simulink model "dcmotor_20240522"  (R2022a)
settings: Solver=ode45  StartTime=0.0  StopTime=1  RelTol=1e-3
values from neighbouring files (symbols this model uses):
  Ce = 1/317    (= 0.00315457413249)    [init_dc_servo.m]
  Cm = 30.2e-3    (= 0.0302)    [init_dc_servo.m]
  J = 142e-7    (= 1.42e-05)    [init_dc_servo.m]
  Kii = 600    [init_dc_servo.m]
  Kip = 2700    [init_dc_servo.m]
  Kpp = 30    [init_dc_servo.m]
  Kvi = 60    [init_dc_servo.m]
  Kvp = 1200    [init_dc_servo.m]
  L = 0.0823e-3    (= 8.23e-05)    [init_dc_servo.m]
  R = 0.299    [init_dc_servo.m]    (also in para_for_math_pmsm.m = 0.958)
libraries: simulink_extras x17, spspowerguiLib x1
settings Model: Creator=ccaao  LastModifiedBy=ccaao

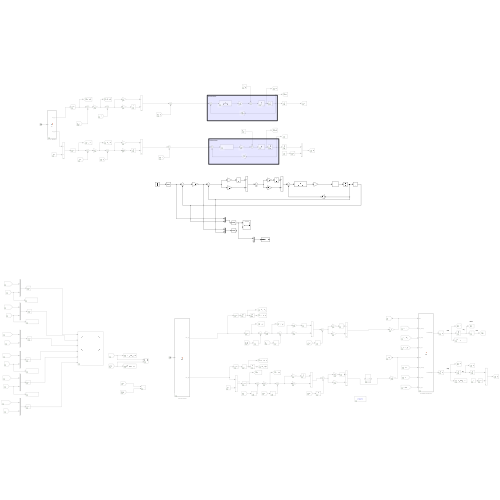
[thumbnail: Simulink's stored preview of the top-level diagram]
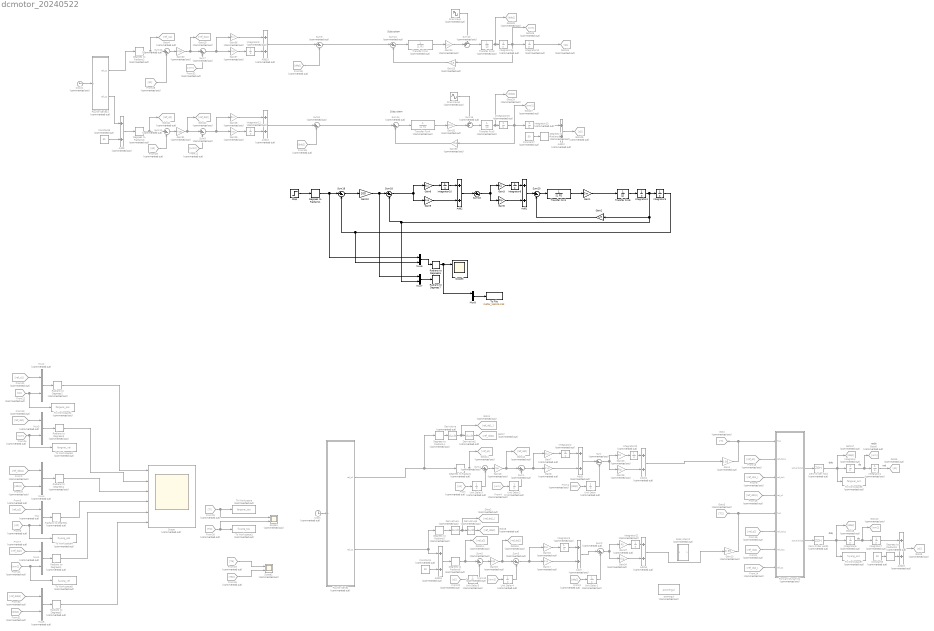
== system dcmotor_20240522 ==
  note: Subsystem
  note: rad/s
  note: rad
  note: dq
  note: ddq
  note: dq
  note: ddq
  note: Subsystem
  Add1 : Sum
  Add{3,7,9..14,18..19} (10 alike) : Sum  Commented=on
  Add2 : Sum
  Clock : Clock  Commented=on
  Clock1 : Clock  Commented=on
  Constant{4..7} (4 alike) : Constant  Commented=on  Value=50
  Degrees to Radians{,2..6,8..9} (8 alike) : simulink_extras/Transformations/Degrees to Radians  Commented=on
  Degrees to Radians1 : simulink_extras/Transformations/Degrees to Radians
  Derivative{,1..3} (4 alike) : Derivative  Commented=on
  Forward Dynamics : MATLAB Function  Commented=on  TreatAsAtomicUnit=on
  Fourier Series : MATLAB Function  Commented=on  TreatAsAtomicUnit=on
  Fourier Series1 : MATLAB Function  Commented=on  TreatAsAtomicUnit=on
  From : From  Commented=on  GotoTag=q1
  From1 : From  Commented=on  GotoTag=ddq1
  From10 : From  Commented=on  GotoTag=wm2
  From11 : From  Commented=on  GotoTag=wm2
  From12 : From  Commented=on  GotoTag=wm2
  From13 : From  Commented=on  GotoTag=ref_q1
  From14 : From  Commented=on  GotoTag=ref_dq2_
  From15 : From  Commented=on  GotoTag=ref_ddq1
  From16 : From  Commented=on  GotoTag=ref_q2
  From19 : From  Commented=on  GotoTag=Te
  From2 : From  Commented=on  GotoTag=ref_ddq1
  From20 : From  Commented=on  GotoTag=q2
  From21 : From  Commented=on  GotoTag=ref_q1
  From22 : From  Commented=on  GotoTag=q1
  From23 : From  Commented=on  GotoTag=ref_dq1
  From24 : From  Commented=on  GotoTag=wm
  From25 : From  Commented=on  GotoTag=Tl
  From26 : From  Commented=on  GotoTag=Tl2
  From27 : From  Commented=on  GotoTag=ddq1
  From28 : From  Commented=on  GotoTag=q1
  From29 : From  Commented=on  GotoTag=q2
  From3 : From  Commented=on  GotoTag=ddq2
  From30 : From  Commented=on  GotoTag=ref_ddq2
  From31 : From  Commented=on  GotoTag=ddq2
  From32 : From  Commented=on  GotoTag=wm
  From35 : From  Commented=on  GotoTag=ddq1
  From36 : From  Commented=on  GotoTag=ddq2
  From4 : From  Commented=on  GotoTag=wm
  From45 : From  Commented=on  GotoTag=Te2
  From5 : From  Commented=on  GotoTag=ref_q2
  From6 : From  Commented=on  GotoTag=q2
  From7 : From  Commented=on  GotoTag=ref_dq2
  From8 : From  Commented=on  GotoTag=ref_dq1_
  From9 : From  Commented=on  GotoTag=ref_dq2
  Gain1 : Gain  Gain=Cm
  Gain10 : Gain  Gain=100
  Gain13 : Gain  Commented=on  Gain=0.95
  Gain{7,16,28,36} (4 alike) : Gain  Commented=on  Gain=Kvi
  Gain{8,17,29,37} (4 alike) : Gain  Commented=on  Gain=Kvp
  Gain{18..19,30..31} (4 alike) : Gain  Commented=on  Gain=Kpp
  Gain2 : Gain  Gain=Ce
  Gain23 : Gain  Commented=on  Gain=Kii
  Gain24 : Gain  Commented=on  Gain=Cm
  Gain25 : Gain  Commented=on  Gain=Ce
  Gain26 : Gain  Commented=on  Gain=Kip
  Gain27 : Gain  Commented=on  Gain=Kii
  Gain3 : Gain  Gain=Kii
  Gain32 : Gain  Commented=on  Gain=Cm
  Gain33 : Gain  Commented=on  Gain=Ce
  Gain34 : Gain  Commented=on  Gain=Kip
  Gain4 : Gain  Commented=on  Gain=0.95
  Gain5 : Gain  Gain=Kip
  Gain6 : Gain  Gain=Kvi
  Gain9 : Gain  Gain=Kvp
  Goto : Goto  Commented=on  GotoTag=Tl
  Goto1 : Goto  Commented=on  GotoTag=ref_dq1_
  Goto10 : Goto  Commented=on  GotoTag=wm2
  Goto11 : Goto  Commented=on  GotoTag=ref_q1
  Goto12 : Goto  Commented=on  GotoTag=ref_dq1
  Goto14 : Goto  Commented=on  GotoTag=ref_q2
  Goto15 : Goto  Commented=on  GotoTag=ref_dq2
  Goto17 : Goto  Commented=on  GotoTag=ddq1
  Goto18 : Goto  Commented=on  GotoTag=ddq2
  Goto19 : Goto  Commented=on  GotoTag=ref_dq1
  Goto2 : Goto  Commented=on  GotoTag=ref_dq2_
  Goto21 : Goto  Commented=on  GotoTag=ref_q2
  Goto22 : Goto  Commented=on  GotoTag=ref_dq2
  Goto24 : Goto  Commented=on  GotoTag=q1
  Goto25 : Goto  Commented=on  GotoTag=q2
  Goto26 : Goto  Commented=on  GotoTag=wm
  Goto27 : Goto  Commented=on  GotoTag=wm2
  Goto28 : Goto  Commented=on  GotoTag=ddq1
  Goto29 : Goto  Commented=on  GotoTag=ddq2
  Goto3 : Goto  Commented=on  GotoTag=Tl2
  Goto4 : Goto  Commented=on  GotoTag=ref_q1
  Goto5 : Goto  Commented=on  GotoTag=q1
  Goto6 : Goto  Commented=on  GotoTag=wm
  Goto7 : Goto  Commented=on  GotoTag=ref_ddq1
  Goto8 : Goto  Commented=on  GotoTag=ref_ddq2
  Goto9 : Goto  Commented=on  GotoTag=q2
  Integrator{,1..3,6..7,9,11..15,20..21} (14 alike) : Integrator  Commented=on
  Integrator{4..5,8,10} (4 alike) : Integrator
  Mux{,1..5} (6 alike) : Mux  Commented=on  Inputs=2
  Mux6 : Mux  Inputs=2
  Mux7 : Mux  Inputs=2
  Mux8 : Mux  Inputs=2
  Radians to Degrees{,1..5} (6 alike) : simulink_extras/Transformations/Radians to Degrees  Commented=on
  Radians to Degrees6 : simulink_extras/Transformations/Radians to Degrees
  Radians to Degrees7 : simulink_extras/Transformations/Radians to Degrees
  Scope : Scope  Commented=on  NumInputPorts=6
  Scope1 : Scope  Commented=on  NumInputPorts=2
  Scope2 : Scope  Commented=on  NumInputPorts=2
  Scope3 : Scope  NumInputPorts=2
  Sine Wave : Sin  Commented=on  Amplitude=10  Frequency=2  SampleTime=0
  Sine Wave1 : Sin  Commented=on  Amplitude=5  SampleTime=0
  Step : Step  Time=0  After=10  SampleTime=0
  Subsystem2 : Subsystem  Commented=on
  Sum{,1..12,14} (14 alike) : Sum  Commented=on  Inputs=|+-
  Sum13 : Sum  Commented=on  Inputs=-+|
  Sum15 : Sum  Commented=on  Inputs=-+|
  Sum{16,18..20} (4 alike) : Sum  Inputs=|+-
  To File : ToFile  Filename=motor_kp0.01.mat
  To Workspace : ToWorkspace  Commented=on  VariableName=fangwei_tau  SampleTime=-1
  To Workspace1 : ToWorkspace  Commented=on  VariableName=fuyang_tau  SampleTime=-1
  To Workspace2 : ToWorkspace  Commented=on  VariableName=fangwei_pos  SampleTime=-1
  To Workspace3 : ToWorkspace  Commented=on  VariableName=fangwei_vel  SampleTime=-1
  To Workspace4 : ToWorkspace  Commented=on  VariableName=fuyang_pos  SampleTime=-1
  To Workspace5 : ToWorkspace  Commented=on  VariableName=fuyang_vel  SampleTime=-1
  To Workspace6 : ToWorkspace  Commented=on  VariableName=fangwei_acc  SampleTime=-1
  To Workspace7 : ToWorkspace  Commented=on  VariableName=fuyang_acc  SampleTime=-1
  Transfer Fcn1 : TransferFcn  Denominator=[L R]
  Transfer Fcn2 : TransferFcn  Commented=on  Denominator=[L R]
  Transfer Fcn3 : TransferFcn  Commented=on  Denominator=[J]
  Transfer Fcn4 : TransferFcn  Commented=on  Denominator=[L R]
  Transfer Fcn5 : TransferFcn  Commented=on  Denominator=[J]
  Transfer Fcn6 : TransferFcn  Denominator=[J]
  Unit Delay{,1..5} (6 alike) : UnitDelay  Commented=on  SampleTime=-1  HasFrameUpgradeWarning=on
  Zero-Order Hold : ZeroOrderHold  Commented=on  SampleTime=0.0005
  Zero-Order Hold1 : ZeroOrderHold  Commented=on  SampleTime=0.0005
  powergui : spspowerguiLib/powergui  Priority=1  Commented=on  SimulationMode=Discrete  SampleTime=0.0005  frequency=60  Iterations=50  frequencyindice=60  Pbase=100e6  ErrMax=1e-4  UnitsV=kV  UnitsW=MW  buscounter=0  FunctionMessages=off  echomessages=off  EnableUseOfTLC=off  CurrentSourceSwitches=off  DisableSnubberDevices=off  DisableRonSwitches=off  DisableVfSwitches=off  DisplayEquations=off  AutomaticDiscreteSolvers=off  SolverType=Tustin/Backward Euler (TBE)  Interpol=off  ExternalGateDelay=off  methode=off  Ts=100  x0status=blocks  SPID=on  SwTol=0  HookPort=off  NonlinearTolerance=1e-4  nMaxIteration=100  ContinueOnMaxIteration=off  RestoreLinks=warning  ResistiveCurrentMeasurement=off  Frange=[0:2:500]  Ylog=off  Xlog=on  ShowGrid=off  save=off  variable=ZData  structure=0  ZoomFFT=off  StartTime=0.0  cycles=1  DisplayStyle=1  fundamental=60  FreqAxis=off  MaxFrequency=1000  frequencyindicesteady=1  RmsSteady=1  display=off
  wires:
  Integrator14/1 -> Goto26/1, Integrator12/1, Gain25/1
  Add11/1 -> Gain4/1
  Integrator/1 -> Goto6/1, Integrator1/1
  Integrator1/1 -> Goto5/1
  Forward Dynamics/1(actualddq1) -> Zero-Order Hold/1
  Sum1/1 -> Gain8/1, Gain7/1
  Gain8/1 -> Add3/2
  Gain7/1 -> Integrator2/1
  Gain16/1 -> Integrator3/1
  Gain17/1 -> Add7/2
  Sum3/1 -> Gain16/1, Gain17/1
  Add14/1 -> Gain13/1
  Integrator6/1 -> Integrator7/1, Goto10/1
  Forward Dynamics/2(actualddq2) -> Zero-Order Hold1/1
  Gain4/1 -> Goto/1, Forward Dynamics/1(Te1)
  Gain13/1 -> Goto3/1, Forward Dynamics/5(Te2)
  Sum4/1 -> Gain18/1
  Sum5/1 -> Gain19/1
  From13/1 -> Forward Dynamics/2(ref_ddq1)
  From8/1 -> Forward Dynamics/3(ref_dq1)
  From15/1 -> Forward Dynamics/4(ref_q1)
  From16/1 -> Forward Dynamics/6(ref_ddq2)
  From9/1 -> Forward Dynamics/7(ref_dq2)
  From14/1 -> Forward Dynamics/8(ref_q2)
  Clock/1 -> Fourier Series/1(t)
  Degrees to Radians/1 -> Goto11/1, Sum4/1
  Add18/1 -> Degrees to Radians6/1
  From5/1 -> Mux/1
  From6/1 -> To Workspace4/1, Mux/2
  Mux/1 -> Radians to Degrees/1
  From7/1 -> Mux1/1
  From12/1 -> To Workspace5/1, Mux1/2
  Mux1/1 -> Radians to Degrees1/1
  Radians to Degrees/1 -> Scope/4
  Radians to Degrees1/1 -> Scope/5
  From21/1 -> Mux2/1
  From22/1 -> To Workspace2/1, Mux2/2
  From23/1 -> Mux3/1
  From24/1 -> To Workspace3/1, Mux3/2
  Mux2/1 -> Radians to Degrees2/1
  Mux3/1 -> Radians to Degrees3/1
  Radians to Degrees2/1 -> Scope/1
  Radians to Degrees3/1 -> Scope/2
  From25/1 -> To Workspace/1, Scope1/1
  From26/1 -> To Workspace1/1, Scope1/2
  Degrees to Radians3/1 -> Goto21/1, Sum11/1
  Degrees to Radians2/1 -> Goto4/1, Sum10/1
  Fourier Series1/1(ref_q1) -> Degrees to Radians2/1
  Clock1/1 -> Fourier Series1/1(t)
  From29/1 -> Sum11/2
  From28/1 -> Sum10/2
  Gain31/1 -> Sum9/1, Goto22/1
  Sum11/1 -> Gain31/1
  Sum10/1 -> Gain30/1
  Gain30/1 -> Goto19/1, Sum7/1
  Sum9/1 -> Gain29/1, Gain28/1
  Integrator11/1 -> Add13/2
  Gain29/1 -> Integrator11/1
  Gain28/1 -> Add13/1
  From11/1 -> Sum9/2
  From32/1 -> Sum7/2
  Gain36/1 -> Add10/1
  Gain37/1 -> Integrator9/1
  Integrator9/1 -> Add10/2
  Sum7/1 -> Gain36/1, Gain37/1
  Sum12/1 -> Transfer Fcn2/1
  Sum13/1 -> Transfer Fcn3/1
  Transfer Fcn2/1 -> Gain24/1
  Gain25/1 -> Sum12/2
  Gain24/1 -> Sum13/2
  Gain32/1 -> Sum15/2
  Gain33/1 -> Sum14/2
  Transfer Fcn4/1 -> Gain32/1
  Sum15/1 -> Transfer Fcn5/1
  Sum14/1 -> Transfer Fcn4/1
  Integrator15/1 -> Goto27/1, Gain33/1, Integrator13/1
  Integrator12/1 -> Goto24/1
  Transfer Fcn3/1 -> Goto28/1, Integrator14/1
  Transfer Fcn5/1 -> Goto29/1, Integrator15/1
  Gain18/1 -> Sum1/1, Goto12/1
  Gain19/1 -> Sum3/1, Goto15/1
  Constant4/1 -> Add18/2
  Integrator7/1 -> Add19/1
  Add19/1 -> Goto9/1
  Constant5/1 -> Degrees to Radians8/1
  Degrees to Radians8/1 -> Add19/2
  From19/1 -> Scope2/1
  From45/1 -> Scope2/2
  Add9/1 -> Degrees to Radians3/1
  Fourier Series1/2(ref_q2) -> Add9/1
  Constant6/1 -> Add9/2
  Integrator13/1 -> Add12/1
  Add12/1 -> Goto25/1
  Degrees to Radians9/1 -> Add12/2
  Constant7/1 -> Degrees to Radians9/1
  Sine Wave/1 -> Sum13/1
  Sine Wave1/1 -> Sum15/1
  From2/1 -> Mux4/1
  From27/1 -> Mux4/2
  Mux4/1 -> Radians to Degrees4/1
  Radians to Degrees4/1 -> Scope/3
  From30/1 -> Mux5/1
  From31/1 -> Mux5/2
  Mux5/1 -> Radians to Degrees5/1
  Radians to Degrees5/1 -> Scope/6
  Integrator2/1 -> Add3/1
  Integrator3/1 -> Add7/1
  Add10/1 -> Sum6/1
  From35/1 -> Sum6/2
  Sum6/1 -> Sum12/1
  Add13/1 -> Sum8/1
  Sum8/1 -> Sum14/1
  From36/1 -> Sum8/2
  Derivative/1 -> Goto1/1, Derivative2/1
  Derivative1/1 -> Goto2/1, Derivative3/1
  Degrees to Radians4/1 -> Derivative/1
  Degrees to Radians5/1 -> Derivative1/1
  Degrees to Radians6/1 -> Goto14/1, Sum5/1
  Integrator20/1 -> Add11/1
  Gain23/1 -> Integrator20/1
  Gain26/1 -> Add11/2
  Add3/1 -> Sum/1
  Sum/1 -> Gain26/1, Gain23/1
  Sum2/1 -> Gain27/1, Gain34/1
  Gain34/1 -> Add14/2
  Gain27/1 -> Integrator21/1
  Integrator21/1 -> Add14/1
  Add7/1 -> Sum2/1
  Derivative2/1 -> Goto7/1
  Derivative3/1 -> Goto8/1
  Zero-Order Hold1/1 -> To Workspace7/1, Goto18/1, Integrator6/1
  Zero-Order Hold/1 -> Goto17/1, To Workspace6/1, Integrator/1
  From20/1 -> Unit Delay5/1
  From10/1 -> Unit Delay4/1
  From3/1 -> Unit Delay1/1
  From1/1 -> Unit Delay/1
  From/1 -> Unit Delay3/1
  From4/1 -> Unit Delay2/1
  Fourier Series/2(ref_q2) -> Add18/1, Degrees to Radians5/1
  Fourier Series/1(ref_q1) -> Degrees to Radians4/1, Degrees to Radians/1
  Unit Delay/1 -> Sum/2
  Unit Delay1/1 -> Sum2/2
  Unit Delay3/1 -> Sum4/2
  Unit Delay2/1 -> Sum1/2
  Unit Delay4/1 -> Sum3/2
  Unit Delay5/1 -> Sum5/2
  Transfer Fcn6/1 -> Integrator4/1
  Gain1/1 -> Transfer Fcn6/1
  Transfer Fcn1/1 -> Gain1/1
  Sum16/1 -> Gain3/1, Gain5/1
  Gain5/1 -> Add1/2
  Gain3/1 -> Integrator8/1
  Integrator8/1 -> Add1/1
  Add2/1 -> Sum16/1
  Integrator10/1 -> Add2/1
  Gain6/1 -> Integrator10/1
  Gain9/1 -> Add2/2
  Sum18/1 -> Gain9/1, Gain6/1
  Gain10/1 -> Mux7/1, Sum18/1
  Sum19/1 -> Gain10/1
  Step/1 -> Degrees to Radians1/1
  Sum20/1 -> Transfer Fcn1/1
  Add1/1 -> Sum20/1
  Gain2/1 -> Sum20/2
  Mux6/1 -> Radians to Degrees6/1
  Mux7/1 -> Radians to Degrees7/1
  Degrees to Radians1/1 -> Mux6/1, Sum19/1
  Radians to Degrees6/1 -> Mux8/1, Scope3/1
  Mux8/1 -> To File/1
  Integrator5/1 -> Mux6/2, Sum19/2
  Integrator4/1 -> Sum18/2, Mux7/2, Gain2/1, Integrator5/1

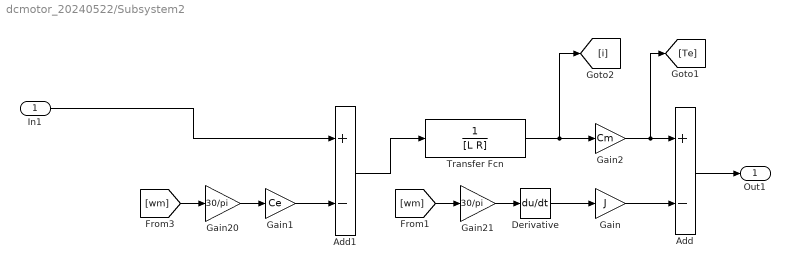
== system dcmotor_20240522/Subsystem2 ==
  In1 : Inport
  Add : Sum  Inputs=+-
  Add1 : Sum  Inputs=+-
  Derivative : Derivative
  Gain : Gain  Gain=J
  Gain1 : Gain  Gain=Ce
  Gain2 : Gain  Gain=Cm
  Gain20 : Gain  Gain=30/pi
  Gain21 : Gain  Gain=30/pi
  Transfer Fcn : TransferFcn  Denominator=[L R]
  Out1 : Outport
  wires:
  Add1/1 -> Transfer Fcn/1
  [wm] -> Gain21/1
  [wm] -> Gain20/1
  Derivative/1 -> Gain/1
  Transfer Fcn/1 -> [i], Gain2/1
  Gain/1 -> Add/2
  Gain2/1 -> [Te], Add/1
  Gain1/1 -> Add1/2
  Gain20/1 -> Gain1/1
  Gain21/1 -> Derivative/1
  Add/1 -> Out1/1
  In1/1 -> Add1/1

== matlab function dcmotor_20240522/Fourier Series ==
  data: t input; ref_q1 output; ref_q2 output
function [ref_q1, ref_q2] = fcn(t)
%%%%%%%%%%%%%%%%%%%%%%%%%%%%%%%%%%%%%%%%%%%%%%%%%%%%%%%%%%%%%%%%%%%%%%%%%%
% 根据输入时间，自动成生成傅里叶轨迹
% input:
%     t - 当前时刻
% outputs:
%     ref_q1 - 方位关节的角位移
%     ref_q2 - 俯仰关节的角位移
%%%%%%%%%%%%%%%%%%%%%%%%%%%%%%%%%%%%%%%%%%%%%%%%%%%%%%%%%%%%%%%%%%%%%%%%%%
A = [-3.146010761462184  -5.024026661537667   4.456211620370575   3.472174388064174   0.241651414565105;
    -6.833423966233333   5.581667583287516   2.791427651070461  -1.733385429140298   0.193714161015655];
B = [0.289573903779656  -0.775328307706171   0.482319175198197  -0.613864619638816   0.453916732918672;
    0.803089511289216  -1.467625820223815  -1.162496361868169   1.038180480795734   0.293385692649764];
N = 5;
w = 0.314159265358979;
q0 = [0;50];
q = zeros(size(q0));
dq = zeros(size(q0));
ddq = zeros(size(q0));

for k = 1:N
   q = q + A(:,k)./(w*k).*sin(w*k*t) - B(:,k)./(w*k).*cos(w*k*t);
   dq = dq + A(:,k).*cos(w*k*t) + B(:,k).*sin(w*k*t);
   ddq = ddq - A(:,k)*w*k.*sin(w*k*t) + B(:,k)*w*k.*cos(w*k*t);
end

ref_q1 = q(1) ;
ref_q2 = q(2) ;

% ref_q1 = dq(1);
% ref_q2 = dq(2);

== matlab function dcmotor_20240522/Forward Dynamics ==
  data: Te1 input; ref_ddq1 input; ref_dq1 input; ref_q1 input; actualddq1 output; Te2 input; ref_ddq2 input; ref_dq2 input; ref_q2 input; actualddq2 output
function [actualddq1,actualddq2] = fcn(Te1, ref_ddq1, ref_dq1, ref_q1, Te2, ref_ddq2, ref_dq2, ref_q2)
%%%%%%%%%%%%%%%%%%%%%%%%%%%%%%%%%%%%%%%%%%%%%%%%%%%%%%%%%%%%
% 天线两个关节的正向动力学模型
% inputs:
%     Te1, Te2 - 输入力矩
%     ref_q1, ref_q2 - 角位移指令值
%     ref_dq1, ref_dq2 - 角速度指令值
%     ref_ddq1, ref_ddq2 - 角加速度指令值
% outputs:
%     actualddq1, actualddq2 - 角加速度实际值
%%%%%%%%%%%%%%%%%%%%%%%%%%%%%%%%%%%%%%%%%%%%%%%%%%%%%%%%%%%%

% %% 参数赋值
g = 9.8;
L1 = 0.132;
r = [560; 700];

% J1 = 1; J2 = 1;
% Izz1 = 8.4425e-08;
% hx1 = -7.6917e-22; hy1 = -7.9176e-22; hz1 = 5.7858e-14;
% Ixx2 = 12.6148; Ixy2 = 0.1568; Ixz2 = 9.2692; Iyy2 = 19.4207; Iyz2 = -0.2213; Izz2 = 6.8396;
% hx2 = -0.7736; hy2 = 0.1433; hz2 = 1.1294;
% m1 = 24.1939; m2 = 1.2811;
% hx2 = hx2/m2; hy2 = hy2/m2; hz2 = hz2/m2;
% fc1 = 104.9022; fc2 = 18.1798;
% fv1 = 73.7219; fv2 = 10.2536;

J1 = 1; J2 = 1;
Ixx1 = 25.1825; Ixy1 = 2.0705e-26; Ixz1 = -1.2035e-21; Iyy1 = 25.1825; Iyz1 = -1.2035e-21; Izz1 = 4.1907e-07;
hx1 = -8.6690e-22; hy1 = -8.6690e-22; hz1 = 6.1121e-14; m1 = 24.2214;

Ixx2 = 12.9287; Ixy2 = 1.1332; Ixz2 = 9.7191; Iyy2 = 20.1602; Iyz2 = -1.4886; Izz2 = 7.5849;
hx2 = -0.7697; hy2 = 0.1465; hz2 = 1.0266; m2 = 0.3266;

fv1 = 106.0643; fv2 = 73.4245;
fc1 = 18.1135 ; fc2 = 10.2673;

q1 = ref_q1; dq1 = ref_dq1; ddq1 = ref_ddq1;
q2 = ref_q2; dq2 = ref_dq2; ddq2 = ref_ddq2;

%% 或者从antenna_obveras
% M = [Ixx2 + Izz1 + Ixy2*sin(2.0*q2) + 1.0*L1^2*m2 + hx1^2*m1 + hy1^2*m1 + 1.0*hy2^2*m2 + hz2^2*m2 - 1.0*Ixx2*cos(q2)^2 + Iyy2*cos(q2)^2 + hx2^2*m2*cos(q2)^2 - 1.0*hy2^2*m2*cos(q2)^2 - 1.0*hx2*hy2*m2*sin(2.0*q2) + 2.0*L1*hx2*m2*cos(q2) - 2.0*L1*hy2*m2*sin(q2),   Iyz2*cos(q2) + Ixz2*sin(q2)  + hz2*cos(q2) + hx2*m2*( -1.0*hz2*sin(q2) ); 
%     cos(q2)*(Iyz2 - 1.0*hy2*hz2*m2) + sin(q2)*(Ixz2 - 1.0*hx2*hz2*m2), m2*hx2^2 + m2*hy2^2 + Izz2];    % 关节惯性矩阵
% C = [Ixy2*dq2*cos(2.0*q2) + 0.5*Ixx2*dq2*sin(2.0*q2) - 0.5*Iyy2*dq2*sin(2.0*q2)  - 0.5*dq2*hx2^2*m2*sin(2.0*q2) + 0.5*dq2*hy2^2*m2*sin(2.0*q2)  - 1.0*dq2*hx2*hy2*m2*cos(2.0*q2) - 1.0*L1*dq2*hy2*m2*cos(q2) - 1.0*L1*dq2*hx2*m2*sin(q2),  Ixy2*dq1*cos(2.0*q2) + 0.5*Ixx2*dq1*sin(2.0*q2) - 0.5*Iyy2*dq1*sin(2.0*q2) + Ixz2*dq2*cos(q2) - 1.0*Iyz2*dq2*sin(q2) - 0.5*dq1*hx2^2*m2*sin(2.0*q2) + 0.5*dq1*hy2^2*m2*sin(2.0*q2) - 1.0*dq1*hx2*hy2*m2*cos(2.0*q2) - 1.0*L1*dq1*hy2*m2*cos(q2) - 1.0*L1*dq1*hx2*m2*sin(q2) - 1.0*dq2*hx2*hz2*m2*cos(q2) + dq2*hy2*hz2*m2*sin(q2); 
%     0.5*Iyy2*dq1*sin(2.0*q2) - 0.5*Ixx2*dq1*sin(2.0*q2) - 1.0*Ixy2*dq1*cos(2.0*q2) + 0.5*dq1*hx2^2*m2*sin(2.0*q2) - 0.5*dq1*hy2^2*m2*sin(2.0*q2) + dq1*hx2*hy2*m2*cos(2.0*q2) + L1*dq1*hy2*m2*cos(q2) + L1*dq1*hx2*m2*sin(q2) ,  0];    % 科氏力项
% G = [0; g*m2*(hx2*cos(q2) - hy2*sin(q2))];    % 重力
% --------------------------------------------------------------------- %
M = [Ixx2 + Izz1 - (Ixx2 - Iyy2)*cos(q2)^2 + Ixy2*sin(2*q2) + m2*L1^2 + 2*hx2*L1*cos(q2) - 2*hy2*L1*sin(q2), Ixz2*sin(q2) + Iyz2*cos(q2);
                                                                                Ixz2*sin(q2) + Iyz2*cos(q2),                       Izz2];    % 惯性矩阵
C = [Ixz2*dq2^2*cos(q2)- Iyz2*dq2^2*sin(q2) - Ixy2*dq1*dq2 + Ixz2*dq1*dq2- Ixy2*dq1*dq2*cos(q2)+ Ixx2*dq1*dq2*(sin(q2) - sin(q2)^3) - Iyy2*dq1*dq2*(sin(q2) - sin(q2)^3)+ 2*Ixy2*dq1*dq2*cos(q2)^2 + 2*Ixy2*dq1*dq2*cos(q2)^3 - Ixz2*dq1*dq2*cos(q2)^2 + (Ixx2*dq1*dq2*sin(2*q2))/2 - (Iyy2*dq1*dq2*sin(2*q2))/2 + (Iyz2*dq1*dq2*sin(2*q2))/2 - L1*dq1*dq2*hy2*cos(q2)^2 - (L1*dq1*dq2*hx2*sin(2*q2))/2 - L1*dq1*dq2*hy2*cos(q2) - L1*dq1*dq2*hx2*sin(q2);
     Ixz2*(dq1*dq2*cos(q2)^2 - dq1*dq2*cos(q2)) + hx2*L1*sin(q2)*dq1^2 + hy2*L1*cos(q2)*dq1^2 + Izz2*dq1*dq2*sin(q2) + Iyz2*(dq1*dq2*sin(q2) - dq1*dq2*cos(q2)*sin(q2))- Ixy2*(dq1^2*cos(q2)^2 - dq1^2*sin(q2)^2) - Ixx2*dq1^2*cos(q2)*sin(q2) + Iyy2*dq1^2*cos(q2)*sin(q2) ];    % 离心力及科氏力矩阵 
G = [                           0; 
     hx2*g*cos(q2) - hy2*g*sin(q2)];    % 重力项
F = [fv1*dq1 + fc1*tanh(50*dq1);
     fv2*dq2 + fc2*tanh(50*dq2)];
% --------------------------------------------------------------------- %

T = [Te1; Te2];
 
actualddq = inv(M)*(T - C - G -F);

actualddq1 = actualddq(1);
actualddq2 = actualddq(2);

== matlab function dcmotor_20240522/Fourier Series1 ==
  data: t input; ref_q1 output; ref_q2 output
function [ref_q1, ref_q2] = fcn(t)
%%%%%%%%%%%%%%%%%%%%%%%%%%%%%%%%%%%%%%%%%%%%%%%%%%%%%%%%%%%%%%%%%%%%%%%%%%
% 根据输入时间，自动成生成傅里叶轨迹
% input:
%     t - 当前时刻
% outputs:
%     ref_q1 - 方位关节的角位移
%     ref_q2 - 俯仰关节的角位移
%%%%%%%%%%%%%%%%%%%%%%%%%%%%%%%%%%%%%%%%%%%%%%%%%%%%%%%%%%%%%%%%%%%%%%%%%%
A = [-3.146010761462184  -5.024026661537667   4.456211620370575   3.472174388064174   0.241651414565105;
    -6.833423966233333   5.581667583287516   2.791427651070461  -1.733385429140298   0.193714161015655];
B = [0.289573903779656  -0.775328307706171   0.482319175198197  -0.613864619638816   0.453916732918672;
    0.803089511289216  -1.467625820223815  -1.162496361868169   1.038180480795734   0.293385692649764];
N = 5;
w = 0.314159265358979;
q0 = [0;50];
q = zeros(size(q0));
dq = zeros(size(q0));
ddq = zeros(size(q0));

for k = 1:N
   q = q + A(:,k)./(w*k).*sin(w*k*t) - B(:,k)./(w*k).*cos(w*k*t);
   dq = dq + A(:,k).*cos(w*k*t) + B(:,k).*sin(w*k*t);
   ddq = ddq - A(:,k)*w*k.*sin(w*k*t) + B(:,k)*w*k.*cos(w*k*t);
end

ref_q1 = q(1);
ref_q2 = q(2);
